simulink library "loco_native_lib"  (R2024b)
settings: Solver=VariableStepAuto  StartTime=0.0  StopTime=10.0  RelTol=1e-3
undefined symbols (not defined in the file): P, PN
libraries: fl_lib x96, nesl_utility x44, $bdroot x21, simulink x2, sdl_lib x1, batteryecm_lib x1
(part 1 of 2)
settings Model: Creator=BillBeverley  LastModifiedBy=BillBeverley

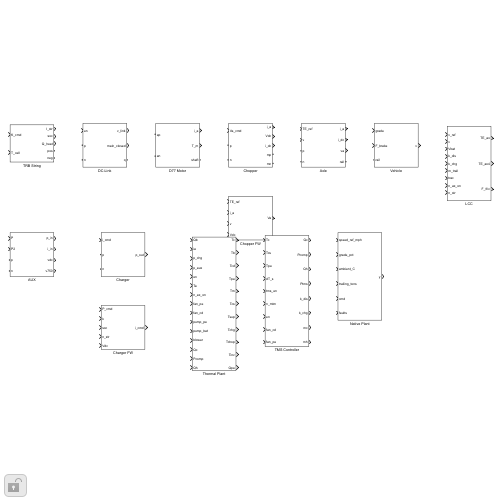
[thumbnail: Simulink's stored preview of the top-level diagram]
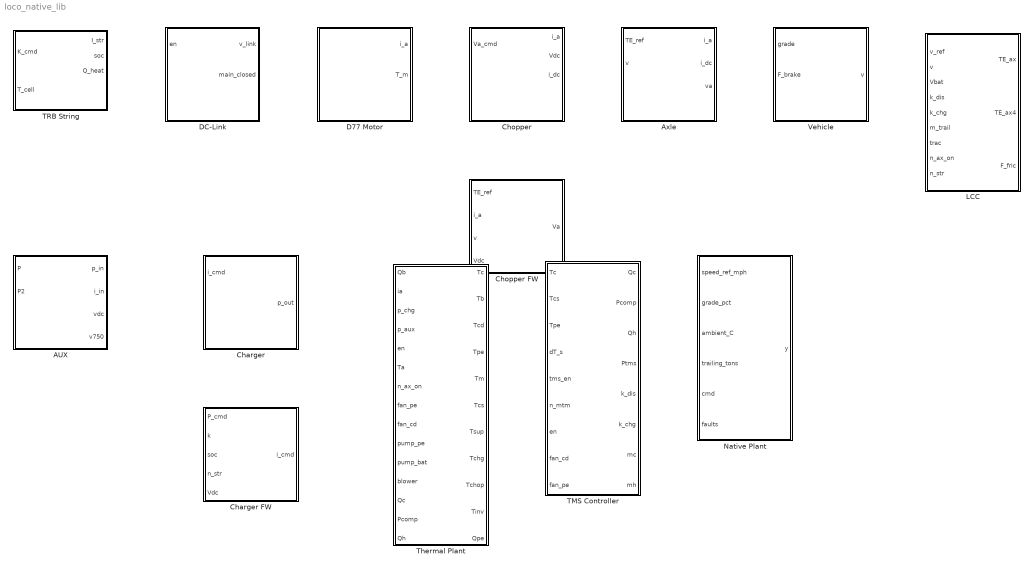
== system loco_native_lib ==
  AUX : Subsystem  mask{eta=P.aux.eta, P_max=P.aux.P_max, V750=750, V_floor=100}
      mask prompts: eta "Converter efficiency"; P_max "Max output power (W)"; V750 "AUX bus voltage (V)"; V_floor "Input voltage floor (V)"
  Axle : Subsystem
  Charger : Subsystem
  Charger FW : Subsystem  mask{P_max=P.chg.P_max, I_max=P.chg.I_hw, I_bms=P.chg.I_bms, soc_max=P.chg.soc_max, soc_band=P.chg.soc_band, V_floor=100, N_str_nom=P.batt.Np, Ts=0.01}
  Chopper : Subsystem
  Chopper FW : Subsystem  mask{A=PN.ax}
      mask prompts: A "Axle parameters (struct)"
  D77 Motor : Subsystem
  DC-Link : Subsystem
  LCC : Subsystem  mask{L=PN.lcc}
      mask prompts: L "LCC parameters (struct)"
  Native Plant : Subsystem
  TMS Controller : Subsystem  mask{TH=P.th, Ts=0.1}
      mask prompts: TH "Thermal parameters (struct)"; Ts "Controller sample time (s)"
  TRB String : Subsystem
  Thermal Plant : Subsystem  mask{TH=P.th, f_ram=0.2}
      mask prompts: TH "Thermal parameters (struct)"; f_ram "Ram-air fraction"
  Vehicle : Subsystem

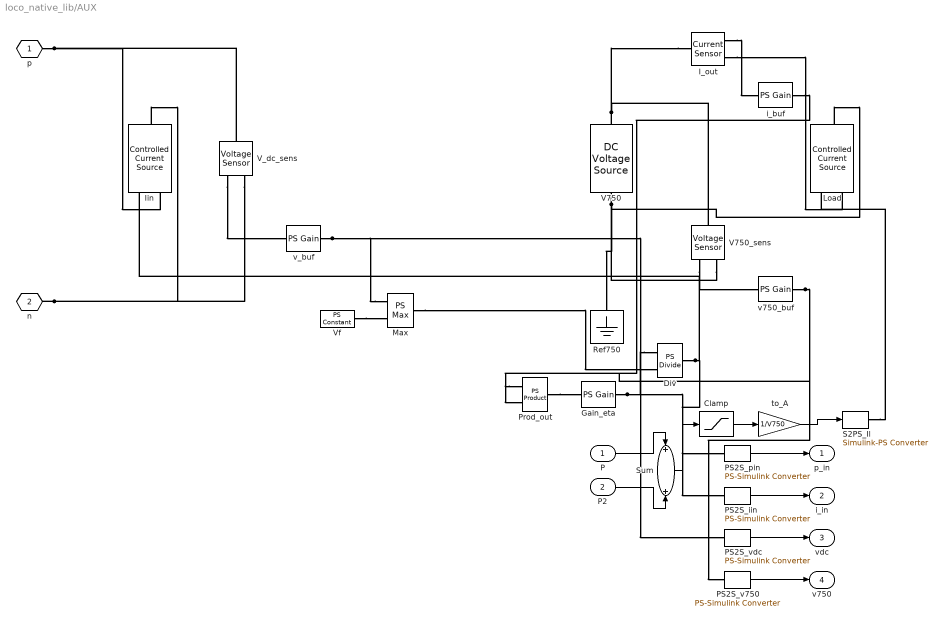
== system loco_native_lib/AUX ==
  P : Inport
  P2 : Inport  Port=2
  Clamp : Saturate  UpperLimit=P_max  LowerLimit=0
  Div : fl_lib/Physical Signals/Functions/PS Divide
  Gain_eta : fl_lib/Physical Signals/Functions/PS Gain  gain=1/eta
  I_out : fl_lib/Electrical/Electrical Sensors/Current Sensor
  Iin : fl_lib/Electrical/Electrical Sources/Controlled Current Source
  Load : fl_lib/Electrical/Electrical Sources/Controlled Current Source
  Max : fl_lib/Physical Signals/Nonlinear Operators/PS Max
      settings: InternalSimscapePortConfiguration="{\"Bottom\":[],\"Left\":[{\"id\":\"I1\",\"label\":\"\",\"type\":\"input\"},{\"id\":\"I2\",\"label\":\"\",\"type\":\"input\"}],\"Right\":[{\"id\":\"O\",\"label\":\"\",\"type\":\"output\"}],\"Top\":[]}"
  PS2S_iin : nesl_utility/PS-Simulink Converter  PhysicalDomain=network_engine_domain  SubClassName=ps_output  LeftPortType=input  RightPortType=output  PseudoPeriodic=off  Frequencies=[]  VectorFormat=inherit  Unit=A  AffineConversion=off
  PS2S_pin : nesl_utility/PS-Simulink Converter  PhysicalDomain=network_engine_domain  SubClassName=ps_output  LeftPortType=input  RightPortType=output  PseudoPeriodic=off  Frequencies=[]  VectorFormat=inherit  Unit=W  AffineConversion=off
  PS2S_v750 : nesl_utility/PS-Simulink Converter  PhysicalDomain=network_engine_domain  SubClassName=ps_output  LeftPortType=input  RightPortType=output  PseudoPeriodic=off  Frequencies=[]  VectorFormat=inherit  Unit=V  AffineConversion=off
  PS2S_vdc : nesl_utility/PS-Simulink Converter  PhysicalDomain=network_engine_domain  SubClassName=ps_output  LeftPortType=input  RightPortType=output  PseudoPeriodic=off  Frequencies=[]  VectorFormat=inherit  Unit=V  AffineConversion=off
  Prod_out : fl_lib/Physical Signals/Functions/PS Product
  Ref750 : fl_lib/Electrical/Electrical Elements/Electrical Reference
  S2PS_Il : nesl_utility/Simulink-PS Converter  PhysicalDomain=network_engine_domain  SubClassName=ps_input  LeftPortType=input  RightPortType=output  PseudoPeriodic=off  Frequencies=[]  NoiseDistribution=none  NoiseParameters=[]  Unit=A  AffineConversion=off  FilteringAndDerivatives=provide  SimscapeFilterOrder=1  InputFilterTimeConstant=0.001  UdotUserProvided=0
  Sum : Sum
  V750 : fl_lib/Electrical/Electrical Sources/DC Voltage Source  v0=V750 V
  V750_sens : fl_lib/Electrical/Electrical Sensors/Voltage Sensor
  V_dc_sens : fl_lib/Electrical/Electrical Sensors/Voltage Sensor
  Vf : fl_lib/Physical Signals/Sources/PS Constant  constant=V_floor V
  i_buf : fl_lib/Physical Signals/Functions/PS Gain  gain=1
  to_A : Gain  Gain=1/V750
  v750_buf : fl_lib/Physical Signals/Functions/PS Gain  gain=1
  v_buf : fl_lib/Physical Signals/Functions/PS Gain  gain=1
  p : PMIOPort  Side=Left
  n : PMIOPort  Port=2  Side=Left
  p_in : Outport
  i_in : Outport  Port=2
  vdc : Outport  Port=3
  v750 : Outport  Port=4
  wires:
  PS2S_pin/1 -> p_in/1
  PS2S_iin/1 -> i_in/1
  PS2S_vdc/1 -> vdc/1
  PS2S_v750/1 -> v750/1
  P/1 -> Sum/1
  P2/1 -> Sum/2
  Sum/1 -> Clamp/1
  Clamp/1 -> to_A/1
  to_A/1 -> S2PS_Il/1
  connections:
  Iin/RConn2 -- p/RConn1 -- V_dc_sens/LConn1
  n/RConn1 -- Iin/LConn1 -- V_dc_sens/RConn2
  I_out/LConn1 -- V750/LConn1 -- V750_sens/LConn1
  I_out/RConn2 -- Load/RConn2
  Load/LConn1 -- Ref750/LConn1 -- V750/RConn1 -- V750_sens/RConn2
  S2PS_Il/RConn1 -- Load/RConn1
  V_dc_sens/RConn1 -- v_buf/LConn1
  V750_sens/RConn1 -- v750_buf/LConn1
  I_out/RConn1 -- i_buf/LConn1
  Iin/RConn1 -- Div/RConn1 -- PS2S_iin/LConn1
  Prod_out/LConn1 -- v750_buf/RConn1 -- PS2S_v750/LConn1
  i_buf/RConn1 -- Prod_out/LConn2
  Prod_out/RConn1 -- Gain_eta/LConn1
  Max/LConn1 -- v_buf/RConn1 -- PS2S_vdc/LConn1
  Vf/RConn1 -- Max/LConn2
  Div/LConn1 -- Gain_eta/RConn1 -- PS2S_pin/LConn1
  Max/RConn1 -- Div/LConn2

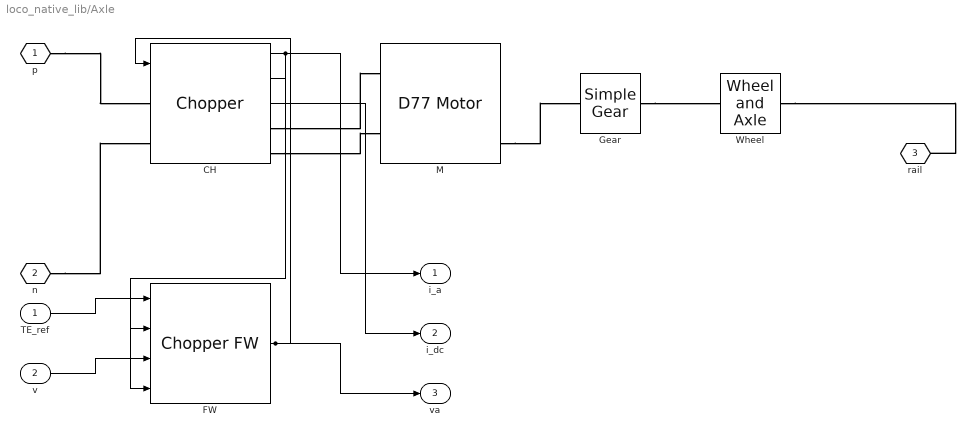
== system loco_native_lib/Axle ==
  TE_ref : Inport
  v : Inport  Port=2
  CH : $bdroot/Chopper  SystemSampleTime=-1  VariantActivationTime=update diagram  AllowFlexibleInterface=on  Latency=0  AutoFrameSizeCalculation=off
  FW : $bdroot/Chopper FW  A=PN.ax
  Gear : sdl_lib/Gears/Simple Gear  ratio=PN.ax.G  rotation_direction=sdl.enum.shaftOutputDirection.same  friction_model=sdl.enum.gear_efficiencies_load.constant  T_noload=0.1 N*m  T_nom=5 N*m  efficiency_nom=0.8  efficiency=PN.ax.eta_g  temperature_TLU=[280, 300, 320] K  load_TLU=[1, 5, 10] N*m  efficiency_TLU=[.95, .9, .85]  efficiency_TLU2=[.85, .8, .75; .95, .9, .85; .85, .8, .7]  w_thr=0.01 rad/s  pwr_thr=1e3 W  enable_backlash=false  hardstop_model=simscape.enum.hardstop.smooth  backlash_distance=1e-3 mm  r_base=0.1 m  transition=1e-4 mm  backlash_stiffness=1e6 N/m  backlash_damping=1e3 N*s/m  coeff_rest=0.7  v_tol=0.001 m/s  f_tol=0.001 N  mu_visc=[0, 0] N*m*s/rad  thermal_mass=50 J/K  temperature_specify=off  temperature_priority=High  temperature=300 K  temperature_nominal_specify=off  temperature_nominal_value=1  temperature_nominal_unit=K  x_backlash_specify=off  x_backlash_priority=None  x_backlash=0 mm  x_backlash_nominal_specify=off  x_backlash_nominal_value=1  x_backlash_nominal_unit=mm  f_hardstop_specify=off  f_hardstop_priority=None  f_hardstop=0 N  f_hardstop_nominal_specify=off  f_hardstop_nominal_value=1  f_hardstop_nominal_unit=N  v_backlash_specify=off  v_backlash_priority=None  v_backlash=0 m/s  v_backlash_nominal_specify=off  v_backlash_nominal_value=1  v_backlash_nominal_unit=m/s
  M : $bdroot/D77 Motor  SystemSampleTime=-1  VariantActivationTime=update diagram  AllowFlexibleInterface=on  Latency=0  AutoFrameSizeCalculation=off
  Wheel : fl_lib/Mechanical/Mechanisms/Wheel and Axle  R=PN.ax.r_w m  or=1  t_specify=off  t_priority=None  t=0 N*m  t_nominal_specify=off  t_nominal_value=1  t_nominal_unit=N*m  f_specify=off  f_priority=None  f=0 N  f_nominal_specify=off  f_nominal_value=1  f_nominal_unit=N
  p : PMIOPort  Side=Left
  n : PMIOPort  Port=2  Side=Left
  rail : PMIOPort  Port=3  Side=Right
  i_a : Outport
  i_dc : Outport  Port=2
  va : Outport  Port=3
  wires:
  TE_ref/1 -> FW/1
  CH/1 -> FW/2, i_a/1
  v/1 -> FW/3
  CH/2 -> FW/4
  FW/1 -> CH/1, va/1
  CH/3 -> i_dc/1
  connections:
  p/RConn1 -- CH/LConn1
  n/RConn1 -- CH/LConn2
  CH/RConn1 -- M/LConn1
  CH/RConn2 -- M/LConn2
  M/RConn1 -- Gear/LConn1
  Gear/RConn1 -- Wheel/LConn1
  Wheel/RConn1 -- rail/RConn1

== system loco_native_lib/Charger ==
  i_cmd : Inport
  Ichg : fl_lib/Electrical/Electrical Sources/Controlled Current Source
  PS2S_p : nesl_utility/PS-Simulink Converter  PhysicalDomain=network_engine_domain  SubClassName=ps_output  LeftPortType=input  RightPortType=output  PseudoPeriodic=off  Frequencies=[]  VectorFormat=inherit  Unit=W  AffineConversion=off
  Prod : fl_lib/Physical Signals/Functions/PS Product
  S2PS_i : nesl_utility/Simulink-PS Converter  PhysicalDomain=network_engine_domain  SubClassName=ps_input  LeftPortType=input  RightPortType=output  PseudoPeriodic=off  Frequencies=[]  NoiseDistribution=none  NoiseParameters=[]  Unit=A  AffineConversion=off  FilteringAndDerivatives=provide  SimscapeFilterOrder=1  InputFilterTimeConstant=0.001  UdotUserProvided=0
  V_sens : fl_lib/Electrical/Electrical Sensors/Voltage Sensor
  p : PMIOPort  Side=Left
  n : PMIOPort  Port=2  Side=Left
  p_out : Outport
  wires:
  i_cmd/1 -> S2PS_i/1
  PS2S_p/1 -> p_out/1
  connections:
  p/RConn1 -- Ichg/LConn1 -- V_sens/LConn1
  n/RConn1 -- Ichg/RConn2 -- V_sens/RConn2
  Ichg/RConn1 -- S2PS_i/RConn1 -- Prod/LConn1
  V_sens/RConn1 -- Prod/LConn2
  Prod/RConn1 -- PS2S_p/LConn1

== system loco_native_lib/Charger FW ==
  P_cmd : Inport
  k : Inport  Port=2
  soc : Inport  Port=3
  n_str : Inport  Port=4
  Vdc : Inport  Port=5
  Mux : Mux  Inputs=5
  Sample : ZeroOrderHold  SampleTime=Ts
  Scan : UnitDelay  SampleTime=Ts  HasFrameUpgradeWarning=on
  chg : MATLAB Function  TreatAsAtomicUnit=on
  i_cmd : Outport
  wires:
  P_cmd/1 -> Mux/1
  k/1 -> Mux/2
  soc/1 -> Mux/3
  n_str/1 -> Mux/4
  Vdc/1 -> Mux/5
  Mux/1 -> Sample/1
  Sample/1 -> chg/1(u)
  chg/1(i) -> Scan/1
  Scan/1 -> i_cmd/1

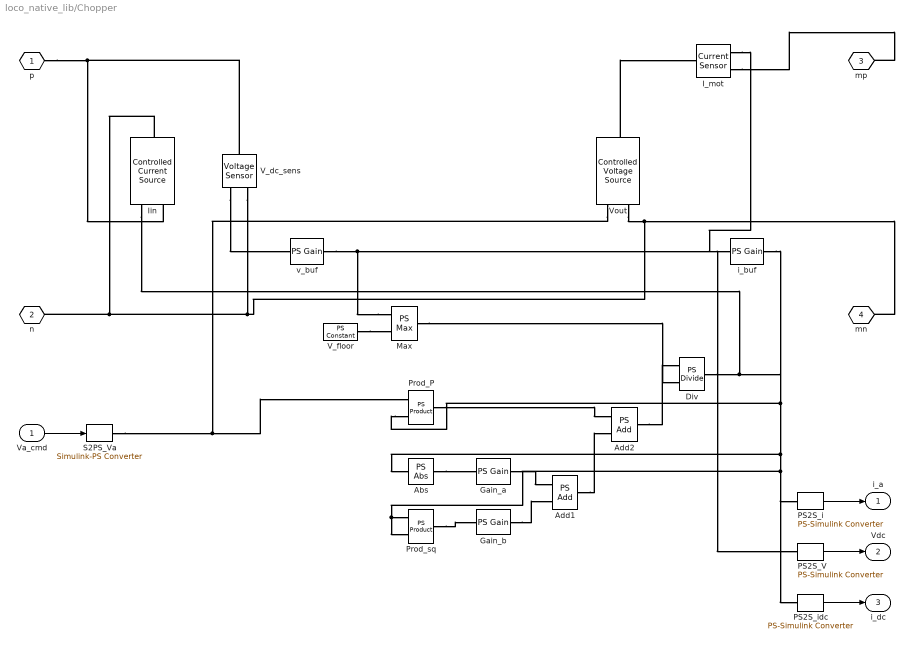
== system loco_native_lib/Chopper ==
  Va_cmd : Inport
  Abs : fl_lib/Physical Signals/Nonlinear Operators/PS Abs
      settings: InternalSimscapePortConfiguration="{\"Bottom\":[],\"Left\":[{\"id\":\"I\",\"label\":\"\",\"type\":\"input\"}],\"Right\":[{\"id\":\"O\",\"label\":\"\",\"type\":\"output\"}],\"Top\":[]}"
  Add1 : fl_lib/Physical Signals/Functions/PS Add
  Add2 : fl_lib/Physical Signals/Functions/PS Add
  Div : fl_lib/Physical Signals/Functions/PS Divide
  Gain_a : fl_lib/Physical Signals/Functions/PS Gain  gain=PN.ax.a_loss V
  Gain_b : fl_lib/Physical Signals/Functions/PS Gain  gain=PN.ax.b_loss Ohm
  I_mot : fl_lib/Electrical/Electrical Sensors/Current Sensor
  Iin : fl_lib/Electrical/Electrical Sources/Controlled Current Source
  Max : fl_lib/Physical Signals/Nonlinear Operators/PS Max
      settings: InternalSimscapePortConfiguration="{\"Bottom\":[],\"Left\":[{\"id\":\"I1\",\"label\":\"\",\"type\":\"input\"},{\"id\":\"I2\",\"label\":\"\",\"type\":\"input\"}],\"Right\":[{\"id\":\"O\",\"label\":\"\",\"type\":\"output\"}],\"Top\":[]}"
  PS2S_V : nesl_utility/PS-Simulink Converter  PhysicalDomain=network_engine_domain  SubClassName=ps_output  LeftPortType=input  RightPortType=output  PseudoPeriodic=off  Frequencies=[]  VectorFormat=inherit  Unit=V  AffineConversion=off
  PS2S_i : nesl_utility/PS-Simulink Converter  PhysicalDomain=network_engine_domain  SubClassName=ps_output  LeftPortType=input  RightPortType=output  PseudoPeriodic=off  Frequencies=[]  VectorFormat=inherit  Unit=A  AffineConversion=off
  PS2S_idc : nesl_utility/PS-Simulink Converter  PhysicalDomain=network_engine_domain  SubClassName=ps_output  LeftPortType=input  RightPortType=output  PseudoPeriodic=off  Frequencies=[]  VectorFormat=inherit  Unit=A  AffineConversion=off
  Prod_P : fl_lib/Physical Signals/Functions/PS Product
  Prod_sq : fl_lib/Physical Signals/Functions/PS Product
  S2PS_Va : nesl_utility/Simulink-PS Converter  PhysicalDomain=network_engine_domain  SubClassName=ps_input  LeftPortType=input  RightPortType=output  PseudoPeriodic=off  Frequencies=[]  NoiseDistribution=none  NoiseParameters=[]  Unit=V  AffineConversion=off  FilteringAndDerivatives=filter  SimscapeFilterOrder=1  InputFilterTimeConstant=1e-4  UdotUserProvided=0
  V_dc_sens : fl_lib/Electrical/Electrical Sensors/Voltage Sensor
  V_floor : fl_lib/Physical Signals/Sources/PS Constant  constant=PN.ax.V_floor V
  Vout : fl_lib/Electrical/Electrical Sources/Controlled Voltage Source
  i_buf : fl_lib/Physical Signals/Functions/PS Gain  gain=1
  v_buf : fl_lib/Physical Signals/Functions/PS Gain  gain=1
  p : PMIOPort  Side=Left
  n : PMIOPort  Port=2  Side=Left
  mp : PMIOPort  Port=3  Side=Right
  mn : PMIOPort  Port=4  Side=Right
  i_a : Outport
  Vdc : Outport  Port=2
  i_dc : Outport  Port=3
  wires:
  Va_cmd/1 -> S2PS_Va/1
  PS2S_i/1 -> i_a/1
  PS2S_V/1 -> Vdc/1
  PS2S_idc/1 -> i_dc/1
  connections:
  S2PS_Va/RConn1 -- Vout/RConn1 -- Prod_P/LConn1
  Prod_P/LConn2 -- i_buf/RConn1 -- Prod_sq/LConn1 -- Prod_sq/LConn2 -- PS2S_i/LConn1 -- Abs/LConn1
  Abs/RConn1 -- Gain_a/LConn1
  Prod_sq/RConn1 -- Gain_b/LConn1
  Gain_a/RConn1 -- Add1/LConn1
  Gain_b/RConn1 -- Add1/LConn2
  Prod_P/RConn1 -- Add2/LConn1
  Add1/RConn1 -- Add2/LConn2
  Max/LConn1 -- v_buf/RConn1 -- PS2S_V/LConn1
  V_floor/RConn1 -- Max/LConn2
  Add2/RConn1 -- Div/LConn1
  Max/RConn1 -- Div/LConn2
  Div/RConn1 -- Iin/RConn1 -- PS2S_idc/LConn1
  p/RConn1 -- V_dc_sens/LConn1 -- Iin/RConn2
  Vout/RConn2 -- n/RConn1 -- Iin/LConn1 -- V_dc_sens/RConn2 -- mn/RConn1
  Vout/LConn1 -- I_mot/LConn1
  I_mot/RConn2 -- mp/RConn1
  I_mot/RConn1 -- i_buf/LConn1
  V_dc_sens/RConn1 -- v_buf/LConn1

== system loco_native_lib/Chopper FW ==
  TE_ref : Inport
  i_a : Inport  Port=2
  v : Inport  Port=3
  Vdc : Inport  Port=4
  Scan : UnitDelay  SampleTime=A.Ts_fw  HasFrameUpgradeWarning=on
  fw : MATLAB Function  TreatAsAtomicUnit=on
  Va : Outport
  wires:
  TE_ref/1 -> fw/1(TE_ref)
  i_a/1 -> fw/2(i_a)
  v/1 -> fw/3(v)
  Vdc/1 -> fw/4(Vdc)
  fw/1(Va) -> Scan/1
  Scan/1 -> Va/1

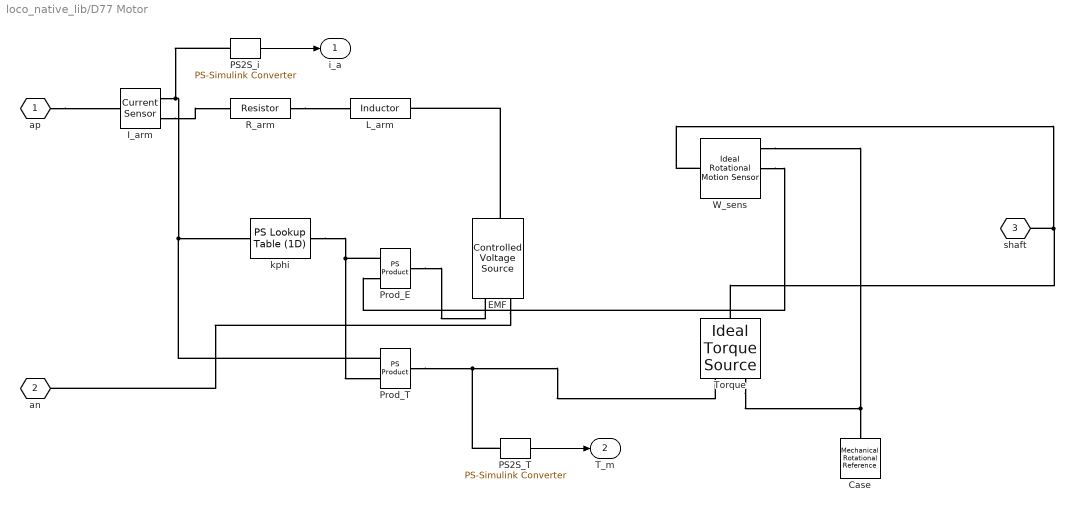
== system loco_native_lib/D77 Motor ==
  Case : fl_lib/Mechanical/Rotational Elements/Mechanical Rotational Reference
  EMF : fl_lib/Electrical/Electrical Sources/Controlled Voltage Source
  I_arm : fl_lib/Electrical/Electrical Sensors/Current Sensor
  L_arm : fl_lib/Electrical/Electrical Elements/Inductor  l=PN.ax.L_a H  r=0 Ohm  g=1e-9 1/Ohm  i_specify=off  i_priority=None  i=0 A  i_nominal_specify=off  i_nominal_value=1  i_nominal_unit=A  v_specify=off  v_priority=None  v=0 V  v_nominal_specify=off  v_nominal_value=1  v_nominal_unit=V  i_L_specify=off  i_L_priority=High  i_L=0 A  i_L_nominal_specify=off  i_L_nominal_value=1  i_L_nominal_unit=A
  PS2S_T : nesl_utility/PS-Simulink Converter  PhysicalDomain=network_engine_domain  SubClassName=ps_output  LeftPortType=input  RightPortType=output  PseudoPeriodic=off  Frequencies=[]  VectorFormat=inherit  Unit=N*m  AffineConversion=off
  PS2S_i : nesl_utility/PS-Simulink Converter  PhysicalDomain=network_engine_domain  SubClassName=ps_output  LeftPortType=input  RightPortType=output  PseudoPeriodic=off  Frequencies=[]  VectorFormat=inherit  Unit=A  AffineConversion=off
  Prod_E : fl_lib/Physical Signals/Functions/PS Product
  Prod_T : fl_lib/Physical Signals/Functions/PS Product
  R_arm : fl_lib/Electrical/Electrical Elements/Resistor  R=PN.ax.R_m Ohm  i_specify=off  i_priority=None  i=0 A  i_nominal_specify=off  i_nominal_value=1  i_nominal_unit=A  v_specify=off  v_priority=None  v=0 V  v_nominal_specify=off  v_nominal_value=1  v_nominal_unit=V
  Torque : fl_lib/Mechanical/Mechanical Sources/Ideal Torque Source
  W_sens : fl_lib/Mechanical/Mechanical Sensors/Ideal Rotational Motion Sensor  reference=foundation.enum.MeasurementReference.difference  acceleration_port=false  velocity_port=true  position_port=true  wrap_angle=false  offset=0 rad
  kphi : fl_lib/Physical Signals/Lookup Tables/PS Lookup Table (1D)  x=PN.ax.i_k A  f=PN.ax.kphi_k V*s/rad  interp_method=simscape.enum.interpolation.linear  extrap_method=simscape.enum.extrapolation.linear
  ap : PMIOPort  Side=Left
  an : PMIOPort  Port=2  Side=Left
  shaft : PMIOPort  Port=3  Side=Right
  i_a : Outport
  T_m : Outport  Port=2
  wires:
  PS2S_i/1 -> i_a/1
  PS2S_T/1 -> T_m/1
  connections:
  ap/RConn1 -- I_arm/LConn1
  I_arm/RConn2 -- R_arm/LConn1
  R_arm/RConn1 -- L_arm/LConn1
  EMF/LConn1 -- L_arm/RConn1
  EMF/RConn2 -- an/RConn1
  Torque/LConn1 -- W_sens/LConn1 -- shaft/RConn1
  Torque/RConn2 -- Case/LConn1 -- W_sens/RConn1
  I_arm/RConn1 -- PS2S_i/LConn1 -- Prod_T/LConn1 -- kphi/LConn1
  kphi/RConn1 -- Prod_E/LConn1 -- Prod_T/LConn2
  W_sens/RConn2 -- Prod_E/LConn2
  Prod_E/RConn1 -- EMF/RConn1
  Prod_T/RConn1 -- PS2S_T/LConn1 -- Torque/RConn1

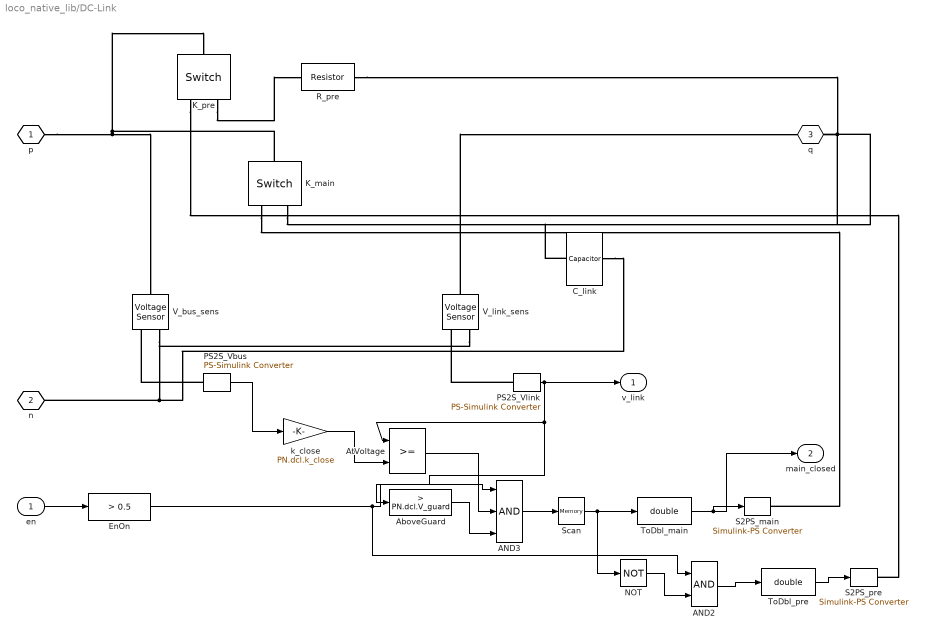
== system loco_native_lib/DC-Link ==
  en : Inport
  AND2 : Logic  AllPortsSameDT=off  OutDataTypeStr=boolean
  AND3 : Logic  Inputs=3  AllPortsSameDT=off  OutDataTypeStr=boolean
  AboveGuard : simulink/Logic and Bit Operations/Compare To Constant  relop=>  const=PN.dcl.V_guard  OutDataTypeStr=boolean
  AtVoltage : RelationalOperator  OutDataTypeStr=boolean  RndMeth=Simplest  InputSameDT=off
  C_link : fl_lib/Electrical/Electrical Elements/Capacitor  c=PN.dcl.C F  r=1e-6 Ohm  g=0 1/Ohm  i_specify=off  i_priority=None  i=0 A  i_nominal_specify=off  i_nominal_value=1  i_nominal_unit=A  v_specify=off  v_priority=None  v=0 V  v_nominal_specify=off  v_nominal_value=1  v_nominal_unit=V  vc_specify=off  vc_priority=High  vc=0 V  vc_nominal_specify=off  vc_nominal_value=1  vc_nominal_unit=V
  EnOn : simulink/Logic and Bit Operations/Compare To Constant  relop=>  const=0.5  OutDataTypeStr=boolean
  K_main : fl_lib/Electrical/Electrical Elements/Switch  R_closed=PN.dcl.R_on Ohm  G_open=1e-9 1/Ohm  Threshold=0.5  i_specify=off  i_priority=None  i=0 A  i_nominal_specify=off  i_nominal_value=1  i_nominal_unit=A  v_specify=off  v_priority=None  v=0 V  v_nominal_specify=off  v_nominal_value=1  v_nominal_unit=V
  K_pre : fl_lib/Electrical/Electrical Elements/Switch  R_closed=PN.dcl.R_pre_k Ohm  G_open=1e-9 1/Ohm  Threshold=0.5  i_specify=off  i_priority=None  i=0 A  i_nominal_specify=off  i_nominal_value=1  i_nominal_unit=A  v_specify=off  v_priority=None  v=0 V  v_nominal_specify=off  v_nominal_value=1  v_nominal_unit=V
  NOT : Logic  Operator=NOT  AllPortsSameDT=off  OutDataTypeStr=boolean
  PS2S_Vbus : nesl_utility/PS-Simulink Converter  PhysicalDomain=network_engine_domain  SubClassName=ps_output  LeftPortType=input  RightPortType=output  PseudoPeriodic=off  Frequencies=[]  VectorFormat=inherit  Unit=V  AffineConversion=off
  PS2S_Vlink : nesl_utility/PS-Simulink Converter  PhysicalDomain=network_engine_domain  SubClassName=ps_output  LeftPortType=input  RightPortType=output  PseudoPeriodic=off  Frequencies=[]  VectorFormat=inherit  Unit=V  AffineConversion=off
  R_pre : fl_lib/Electrical/Electrical Elements/Resistor  R=PN.dcl.R_pre Ohm  i_specify=off  i_priority=None  i=0 A  i_nominal_specify=off  i_nominal_value=1  i_nominal_unit=A  v_specify=off  v_priority=None  v=0 V  v_nominal_specify=off  v_nominal_value=1  v_nominal_unit=V
  S2PS_main : nesl_utility/Simulink-PS Converter  PhysicalDomain=network_engine_domain  SubClassName=ps_input  LeftPortType=input  RightPortType=output  PseudoPeriodic=off  Frequencies=[]  NoiseDistribution=none  NoiseParameters=[]  Unit=1  AffineConversion=off  FilteringAndDerivatives=provide  SimscapeFilterOrder=1  InputFilterTimeConstant=0.001  UdotUserProvided=0
  S2PS_pre : nesl_utility/Simulink-PS Converter  PhysicalDomain=network_engine_domain  SubClassName=ps_input  LeftPortType=input  RightPortType=output  PseudoPeriodic=off  Frequencies=[]  NoiseDistribution=none  NoiseParameters=[]  Unit=1  AffineConversion=off  FilteringAndDerivatives=provide  SimscapeFilterOrder=1  InputFilterTimeConstant=0.001  UdotUserProvided=0
  Scan : Memory
  ToDbl_main : DataTypeConversion  OutDataTypeStr=double  SaturateOnIntegerOverflow=off  RndMeth=Floor
  ToDbl_pre : DataTypeConversion  OutDataTypeStr=double  SaturateOnIntegerOverflow=off  RndMeth=Floor
  V_bus_sens : fl_lib/Electrical/Electrical Sensors/Voltage Sensor
  V_link_sens : fl_lib/Electrical/Electrical Sensors/Voltage Sensor
  k_close : Gain  Gain=PN.dcl.k_close
  p : PMIOPort  Side=Left
  n : PMIOPort  Port=2  Side=Left
  q : PMIOPort  Port=3  Side=Right
  v_link : Outport
  main_closed : Outport  Port=2
  wires:
  en/1 -> EnOn/1
  EnOn/1 -> AND3/1, AND2/1
  PS2S_Vlink/1 -> AtVoltage/1, AboveGuard/1, v_link/1
  PS2S_Vbus/1 -> k_close/1
  k_close/1 -> AtVoltage/2
  AtVoltage/1 -> AND3/2
  AboveGuard/1 -> AND3/3
  AND3/1 -> Scan/1
  Scan/1 -> ToDbl_main/1, NOT/1
  ToDbl_main/1 -> S2PS_main/1, main_closed/1
  NOT/1 -> AND2/2
  AND2/1 -> ToDbl_pre/1
  ToDbl_pre/1 -> S2PS_pre/1
  connections:
  R_pre/RConn1 -- q/RConn1 -- K_main/RConn2 -- V_link_sens/LConn1 -- C_link/LConn1
  p/RConn1 -- V_bus_sens/LConn1 -- K_main/LConn1 -- K_pre/LConn1
  K_pre/RConn2 -- R_pre/LConn1
  C_link/RConn1 -- V_link_sens/RConn2 -- V_bus_sens/RConn2 -- n/RConn1
  K_pre/RConn1 -- S2PS_pre/RConn1
  K_main/RConn1 -- S2PS_main/RConn1
  PS2S_Vlink/LConn1 -- V_link_sens/RConn1
  PS2S_Vbus/LConn1 -- V_bus_sens/RConn1

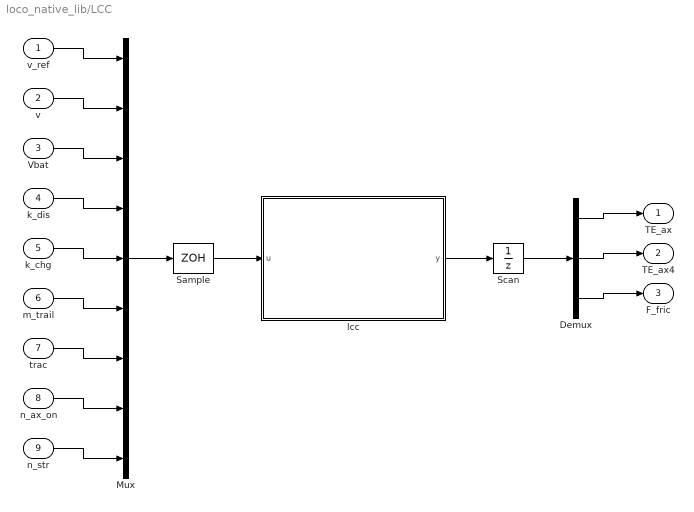
== system loco_native_lib/LCC ==
  v_ref : Inport
  v : Inport  Port=2
  Vbat : Inport  Port=3
  k_dis : Inport  Port=4
  k_chg : Inport  Port=5
  m_trail : Inport  Port=6
  trac : Inport  Port=7
  n_ax_on : Inport  Port=8
  n_str : Inport  Port=9
  Demux : Demux  Outputs=3
  Mux : Mux  Inputs=9
  Sample : ZeroOrderHold  SampleTime=PN.lcc.Ts
  Scan : UnitDelay  SampleTime=PN.lcc.Ts  HasFrameUpgradeWarning=on
  lcc : MATLAB Function  TreatAsAtomicUnit=on
  TE_ax : Outport
  TE_ax4 : Outport  Port=2
  F_fric : Outport  Port=3
  wires:
  v_ref/1 -> Mux/1
  v/1 -> Mux/2
  Vbat/1 -> Mux/3
  k_dis/1 -> Mux/4
  k_chg/1 -> Mux/5
  m_trail/1 -> Mux/6
  trac/1 -> Mux/7
  n_ax_on/1 -> Mux/8
  n_str/1 -> Mux/9
  Mux/1 -> Sample/1
  Sample/1 -> lcc/1(u)
  lcc/1(y) -> Scan/1
  Scan/1 -> Demux/1
  Demux/1 -> TE_ax/1
  Demux/2 -> TE_ax4/1
  Demux/3 -> F_fric/1

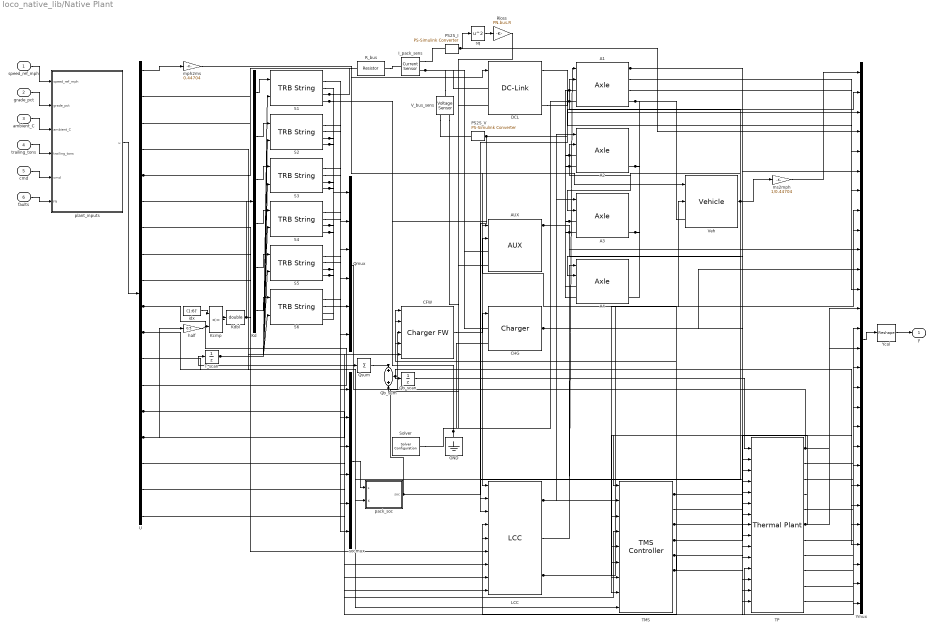
== system loco_native_lib/Native Plant ==
  speed_ref_mph : Inport
  grade_pct : Inport  Port=2
  ambient_C : Inport  Port=3
  trailing_tons : Inport  Port=4
  cmd : Inport  Port=5
  faults : Inport  Port=6
  A{1..4} (4 alike) : $bdroot/Axle  SystemSampleTime=-1  VariantActivationTime=update diagram  AllowFlexibleInterface=on  Latency=0  AutoFrameSizeCalculation=off
  AUX : $bdroot/AUX  eta=P.aux.eta  P_max=P.aux.P_max  V750=750  V_floor=100
  CFW : $bdroot/Charger FW  P_max=P.chg.P_max  I_max=P.chg.I_hw  I_bms=P.chg.I_bms  soc_max=P.chg.soc_max  soc_band=P.chg.soc_band  V_floor=100  N_str_nom=P.batt.Np  Ts=0.01
  CHG : $bdroot/Charger  SystemSampleTime=-1  VariantActivationTime=update diagram  AllowFlexibleInterface=on  Latency=0  AutoFrameSizeCalculation=off
  DCL : $bdroot/DC-Link  SystemSampleTime=-1  VariantActivationTime=update diagram  AllowFlexibleInterface=on  Latency=0  AutoFrameSizeCalculation=off
  GND : fl_lib/Electrical/Electrical Elements/Electrical Reference
  I_pack_sens : fl_lib/Electrical/Electrical Sensors/Current Sensor
  Kcmp : RelationalOperator  Operator=<=  OutDataTypeStr=boolean  RndMeth=Simplest  InputSameDT=off
  Kd : Demux  Outputs=6
  Kdbl : DataTypeConversion  OutDataTypeStr=double  SaturateOnIntegerOverflow=off  RndMeth=Floor
  LCC : $bdroot/LCC  L=PN.lcc
  PS2S_I : nesl_utility/PS-Simulink Converter  PhysicalDomain=network_engine_domain  SubClassName=ps_output  LeftPortType=input  RightPortType=output  PseudoPeriodic=off  Frequencies=[]  VectorFormat=inherit  Unit=A  AffineConversion=off
  PS2S_V : nesl_utility/PS-Simulink Converter  PhysicalDomain=network_engine_domain  SubClassName=ps_output  LeftPortType=input  RightPortType=output  PseudoPeriodic=off  Frequencies=[]  VectorFormat=inherit  Unit=V  AffineConversion=off
  Qb_scan : UnitDelay  SampleTime=0.1  HasFrameUpgradeWarning=on
  Qb_sum : Sum
  Qmux : Mux  Inputs=6
  Qsum : Sum  Inputs=+
  R_bus : fl_lib/Electrical/Electrical Elements/Resistor  R=PN.bus.R Ohm  i_specify=off  i_priority=None  i=0 A  i_nominal_specify=off  i_nominal_value=1  i_nominal_unit=A  v_specify=off  v_priority=None  v=0 V  v_nominal_specify=off  v_nominal_value=1  v_nominal_unit=V
  Rloss : Gain  Gain=PN.bus.R
  S{1..6} (6 alike) : $bdroot/TRB String  SystemSampleTime=-1  VariantActivationTime=update diagram  AllowFlexibleInterface=on  Latency=0  AutoFrameSizeCalculation=off
  Solver : nesl_utility/Solver Configuration  PhysicalDomain=network_engine_domain  SubClassName=solver  LeftPortType=input  RightPortType=generic  Tones=[]  Harmonics=[]  SimulateNoise=off  Profile=off  UseLocalSampling=off  EnableSwitchedLinearOptims=on  FrequencyDomain=off  UseCCode=off  RelTol=0.001  AbsTol=0.001  MinStep=1e-09  ToWorkspace=off  RevertToSquareIcSolve=off  NumHomotopyIterations=100  PhasorMode=off  PhasorModeNumHarmonics=1  ConsistencySolver=NEWTON_XTOL_AFTER_FTOL  IndexReductionMethod=DerivativeReplacement  DoDC=off  ResidualTolerance=1e-09  ConsistencyTolSource=GLOBAL  ConsistencyAbsTol=0.001  ConsistencyRelTol=0.001  ConsistencyTolFactor=0.001  UseLocalSolver=off  LocalSolverChoice=NE_BACKWARD_EULER_ADVANCER  ResolveIndetEquations=on  FunctionEvalNumThread=1  LocalSolverSampleTime=0.001  DoFixedCost=off  MaxNonlinIter=3  MaxModeIter=2  ComputeImpulses=off  ImpulseIterations=2  LinearAlgebra=auto  LinearAlgebraNumThread=0  EquationFormulation=NE_TIME_EF  DelaysMemoryBudget=1024  AutomaticFiltering=on  FilteringTimeConstant=0.001  PartitionStorageMethod=AS_NEEDED  PartitionMemoryBudget=1024  PartitionMethod=ROBUST  MultibodyUseLocalSolver=off  MultibodyLocalSolverChoice=ODE1  MultibodyLocalSolverSampleTime=0.001
  TMS : $bdroot/TMS Controller  TH=P.th  Ts=0.1
  TP : $bdroot/Thermal Plant  TH=P.th  f_ram=0.2
  T_scan : UnitDelay  InitialCondition=P.th.T0_bat  SampleTime=0.1  HasFrameUpgradeWarning=on
  U : Demux  Outputs=18
  V_bus_sens : fl_lib/Electrical/Electrical Sensors/Voltage Sensor
  Veh : $bdroot/Vehicle  SystemSampleTime=-1  VariantActivationTime=update diagram  AllowFlexibleInterface=on  Latency=0  AutoFrameSizeCalculation=off
  Ycol : Reshape  OutputDimensionality=Column vector (2-D)
  Ymux : Mux  Inputs=28
  half : Gain  Gain=0.5
  idx : Constant  Value=(1:6)'
  mph2ms : Gain  Gain=0.44704
  ms2mph : Gain  Gain=1/0.44704
  pack_soc : MATLAB Function  TreatAsAtomicUnit=on
  plant_inputs : MATLAB Function  TreatAsAtomicUnit=on
  socmux : Mux  Inputs=6
  sq : Math  Operator=square
  y : Outport
  wires:
  speed_ref_mph/1 -> plant_inputs/1(speed_ref_mph)
  grade_pct/1 -> plant_inputs/2(grade_pct)
  ambient_C/1 -> plant_inputs/3(ambient_C)
  trailing_tons/1 -> plant_inputs/4(trailing_tons)
  cmd/1 -> plant_inputs/5(cmd)
  faults/1 -> plant_inputs/6(flt)
  plant_inputs/1(u) -> U/1
  U/1 -> mph2ms/1
  mph2ms/1 -> LCC/1
  Veh/1 -> LCC/2, ms2mph/1, A1/2, A2/2, A3/2, A4/2
  PS2S_V/1 -> LCC/3, CFW/5, Ymux/3
  TMS/5 -> LCC/4, Ymux/27
  TMS/6 -> LCC/5, CFW/2, Ymux/28
  U/7 -> LCC/6
  U/18 -> LCC/7
  U/14 -> LCC/8, TP/7
  U/15 -> LCC/9, CFW/4, half/1
  LCC/1 -> A1/1, A2/1, A3/1, Ymux/8
  LCC/2 -> A4/1
  LCC/3 -> Veh/2, Ymux/9
  U/2 -> Veh/1
  U/5 -> DCL/1, TP/5, TMS/7
  U/3 -> AUX/1
  TMS/4 -> AUX/2, Ymux/22
  U/4 -> CFW/1
  pack_soc/1(soc) -> CFW/3, Ymux/2
  CFW/1 -> CHG/1
  Qb_scan/1 -> TP/1
  A1/1 -> TP/2, Ymux/6
  CHG/1 -> TP/3, Ymux/11
  AUX/1 -> TP/4, Ymux/10
  U/6 -> TP/6
  U/10 -> TP/8, TMS/9
  U/11 -> TP/9, TMS/8
  U/12 -> TP/10
  U/13 -> TP/11
  U/17 -> TP/12
  TMS/1 -> TP/13, Ymux/23
  TMS/2 -> TP/14
  TMS/3 -> TP/15, Ymux/24
  TP/1 -> TMS/1, T_scan/1, Ymux/13
  TP/6 -> TMS/2, Ymux/15
  TP/4 -> TMS/3
  U/16 -> TMS/4
  U/8 -> TMS/5
  U/9 -> TMS/6
  idx/1 -> Kcmp/1
  half/1 -> Kcmp/2
  Kcmp/1 -> Kdbl/1
  Kdbl/1 -> Kd/1, pack_soc/2(K)
  socmux/1 -> pack_soc/1(s)
  Qmux/1 -> Qsum/1
  Qsum/1 -> Qb_sum/1
  PS2S_I/1 -> sq/1, Ymux/4
  sq/1 -> Rloss/1
  Rloss/1 -> Qb_sum/2
  Qb_sum/1 -> Qb_scan/1, Ymux/25
  Ymux/1 -> Ycol/1
  Ycol/1 -> y/1
  Kd/1 -> S1/1
  T_scan/1 -> S1/2, S2/2, S3/2, S4/2, S5/2, S6/2
  S1/3 -> Qmux/1
  S1/2 -> socmux/1
  Kd/2 -> S2/1
  S2/3 -> Qmux/2
  S2/2 -> socmux/2
  Kd/3 -> S3/1
  S3/3 -> Qmux/3
  S3/2 -> socmux/3
  Kd/4 -> S4/1
  S4/3 -> Qmux/4
  S4/2 -> socmux/4
  Kd/5 -> S5/1
  S5/3 -> Qmux/5
  S5/2 -> socmux/5
  Kd/6 -> S6/1
  S6/3 -> Qmux/6
  S6/2 -> socmux/6
  ms2mph/1 -> Ymux/1
  DCL/1 -> Ymux/5
  A1/3 -> Ymux/7
  A1/2 -> Ymux/12
  TP/2 -> Ymux/14
  TP/3 -> Ymux/16
  TP/7 -> Ymux/17
  TP/8 -> Ymux/18
  TP/9 -> Ymux/19
  TP/10 -> Ymux/20
  TP/5 -> Ymux/21
  TP/11 -> Ymux/26
  connections:
  R_bus/LConn1 -- S1/RConn1 -- S2/RConn1 -- S3/RConn1 -- S4/RConn1 -- S5/RConn1 -- S6/RConn1
  R_bus/RConn1 -- I_pack_sens/LConn1
  V_bus_sens/LConn1 -- I_pack_sens/RConn2 -- DCL/LConn1 -- AUX/LConn1 -- CHG/LConn1
  V_bus_sens/RConn2 -- S1/RConn2 -- S2/RConn2 -- S3/RConn2 -- S4/RConn2 -- S5/RConn2 -- S6/RConn2 -- DCL/LConn2 -- AUX/LConn2 -- CHG/LConn2 -- Solver/RConn1 -- GND/LConn1 -- A1/LConn2 -- A2/LConn2 -- A3/LConn2 -- A4/LConn2
  I_pack_sens/RConn1 -- PS2S_I/LConn1
  V_bus_sens/RConn1 -- PS2S_V/LConn1
  A1/LConn1 -- DCL/RConn1 -- A2/LConn1 -- A3/LConn1 -- A4/LConn1
  Veh/LConn1 -- A1/RConn1 -- A2/RConn1 -- A3/RConn1 -- A4/RConn1

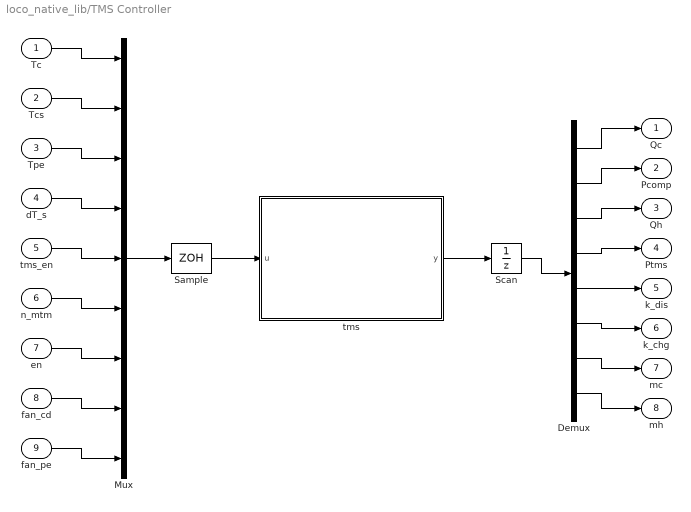
== system loco_native_lib/TMS Controller ==
  Tc : Inport
  Tcs : Inport  Port=2
  Tpe : Inport  Port=3
  dT_s : Inport  Port=4
  tms_en : Inport  Port=5
  n_mtm : Inport  Port=6
  en : Inport  Port=7
  fan_cd : Inport  Port=8
  fan_pe : Inport  Port=9
  Demux : Demux  Outputs=8
  Mux : Mux  Inputs=9
  Sample : ZeroOrderHold  SampleTime=Ts
  Scan : UnitDelay  SampleTime=Ts  HasFrameUpgradeWarning=on
  tms : MATLAB Function  TreatAsAtomicUnit=on
  Qc : Outport
  Pcomp : Outport  Port=2
  Qh : Outport  Port=3
  Ptms : Outport  Port=4
  k_dis : Outport  Port=5
  k_chg : Outport  Port=6
  mc : Outport  Port=7
  mh : Outport  Port=8
  wires:
  Tc/1 -> Mux/1
  Tcs/1 -> Mux/2
  Tpe/1 -> Mux/3
  dT_s/1 -> Mux/4
  tms_en/1 -> Mux/5
  n_mtm/1 -> Mux/6
  en/1 -> Mux/7
  fan_cd/1 -> Mux/8
  fan_pe/1 -> Mux/9
  Mux/1 -> Sample/1
  Sample/1 -> tms/1(u)
  tms/1(y) -> Scan/1
  Scan/1 -> Demux/1
  Demux/1 -> Qc/1
  Demux/2 -> Pcomp/1
  Demux/3 -> Qh/1
  Demux/4 -> Ptms/1
  Demux/5 -> k_dis/1
  Demux/6 -> k_chg/1
  Demux/7 -> mc/1
  Demux/8 -> mh/1

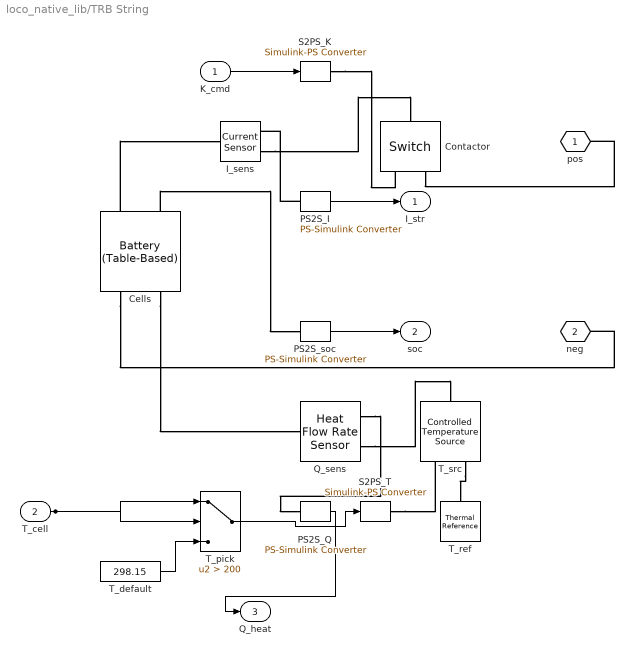
== system loco_native_lib/TRB String ==
  K_cmd : Inport
  T_cell : Inport  Port=2
  Cells : batteryecm_lib/Battery (Table-Based)  SOC_vec=PN.SOC  T_dependence=simscape.enum.tablebattery.temperature_dependence.yes  prm_dir=simscape.enum.tablebattery.prm_dir.noCurrentDirectionality  T_vec=PN.T K  V0_mat=PN.str.V0 V  V0_vec=[3.5057, 3.566, 3.6337, 3.7127, 3.9259, 4.0777, 4.1928] V  V_range=[0 inf] V  R0_mat=PN.str.R0 Ohm  R0_vec=[.0085, .0085, .0087, .0082, .0083, .0085, .0085] Ohm  R0_dis_mat=[.0117, .0085, .009; .011, .0085, .009; .0114, .0087, .0092; .0107, .0082, .0088; .0107, .0083, .0091; .0113, .0085, .0089; .0116, .0085, .0089] Ohm  R0_dis_vec=[.0085, .0085, .0087, .0082, .0083, .0085, .0085] Ohm  R0_ch_mat=[.0117, .0085, .009; .011, .0085, .009; .0114, .0087, .0092; .0107, .0082, .0088; .0107, .0083, .0091; .0113, .0085, .0089; .0116, .0085, .0089] Ohm  R0_ch_vec=[.0085, .0085, .0087, .0082, .0083, .0085, .0085] Ohm  AH=PN.str.Q_Ah A*hr  prm_leak=simscape.enum.tablebattery.prm_leak.disabled  Rleak_vec=[8000, 7000, 6000] Ohm  Rleak=7e3 Ohm  extrapolation_option=simscape.enum.extrapolation.nearest  SOC_port=simscape.enum.tablebattery.enable.yes  prm_dyn=simscape.enum.tablebattery.prm_dyn.rc1  R1_mat=PN.str.R1 Ohm  R1_vec=[.0029, .0024, .0026, .0016, .0023, .0018, .0017] Ohm  tau1_mat=PN.str.tau1 s  tau1_vec=[36, 45, 105, 29, 77, 33, 39] s  R2_mat=[.0109, .0029, .0013; .0069, .0024, .0012; .0047, .0026, .0013; .0034, .0016, .001; .0033, .0023, .0014; .0033, .0018, .0011; .0028, .0017, .0011] Ohm  R2_vec=[.0029, .0024, .0026, .0016, .0023, .0018, .0017] Ohm  tau2_mat=[20, 36, 39; 31, 45, 39; 109, 105, 61; 36, 29, 26; 59, 77, 67; 40, 33, 29; 25, 39, 33] s  tau2_vec=[36, 45, 105, 29, 77, 33, 39] s  R3_mat=[.0109, .0029, .0013; .0069, .0024, .0012; .0047, .0026, .0013; .0034, .0016, .001; .0033, .0023, .0014; .0033, .0018, .0011; .0028, .0017, .0011] Ohm  R3_vec=[.0029, .0024, .0026, .0016, .0023, .0018, .0017] Ohm  tau3_mat=[20, 36, 39; 31, 45, 39; 109, 105, 61; 36, 29, 26; 59, 77, 67; 40, 33, 29; 25, 39, 33] s  tau3_vec=[36, 45, 105, 29, 77, 33, 39] s  R4_mat=[.0109, .0029, .0013; .0069, .0024, .0012; .0047, .0026, .0013; .0034, .0016, .001; .0033, .0023, .0014; .0033, .0018, .0011; .0028, .0017, .0011] Ohm  R4_vec=[.0029, .0024, .0026, .0016, .0023, .0018, .0017] Ohm  tau4_mat=[20, 36, 39; 31, 45, 39; 109, 105, 61; 36, 29, 26; 59, 77, 67; 40, 33, 29; 25, 39, 33] s  tau4_vec=[36, 45, 105, 29, 77, 33, 39] s  R5_mat=[.0109, .0029, .0013; .0069, .0024, .0012; .0047, .0026, .0013; .0034, .0016, .001; .0033, .0023, .0014; .0033, .0018, .0011; .0028, .0017, .0011] Ohm  R5_vec=[.0029, .0024, .0026, .0016, .0023, .0018, .0017] Ohm  tau5_mat=[20, 36, 39; 31, 45, 39; 109, 105, 61; 36, 29, 26; 59, 77, 67; 40, 33, 29; 25, 39, 33] s  tau5_vec=[36, 45, 105, 29, 77, 33, 39] s  prm_fade=simscape.enum.tablebattery.prm_fade.disabled  N0=100  dV0=0  dR0=0  dAH=0  dRleak=0  dR1=0  dR2=0  dR3=0  dR4=0  dR5=0  N0vec=[0, 100, 200, 300]  Tfadevec=[298.15, 323.15] K  dV0vec=[0, 0, 0, 0]  dR0vec=[0, 0, 0, 0]  dAHvec=[0, 0, 0, 0]  dRleakvec=[0, 0, 0, 0]  dR1vec=[0, 0, 0, 0]  dR2vec=[0, 0, 0, 0]  dR3vec=[0, 0, 0, 0]  dR4vec=[0, 0, 0, 0]  dR5vec=[0, 0, 0, 0]  dV0mat=[0, 0; 0, 0; 0, 0; 0, 0]  dR0mat=[0, 0; 0, 0; 0, 0; 0, 0]  dAHmat=[0, 0; 0, 0; 0, 0; 0, 0]  dRleakmat=[0, 0; 0, 0; 0, 0; 0, 0]  dR1mat=[0, 0; 0, 0; 0, 0; 0, 0]  dR2mat=[0, 0; 0, 0; 0, 0; 0, 0]  dR3mat=[0, 0; 0, 0; 0, 0; 0, 0]  dR4mat=[0, 0; 0, 0; 0, 0; 0, 0]  dR5mat=[0, 0; 0, 0; 0, 0; 0, 0]  prm_age_modeling=simscape.enum.tablebattery.prm_age_modeling.equation  storage_dt_age_vec=[0] d  storage_T_age_vec=[273] K  prm_age_OCV=simscape.enum.tablebattery.prm_age_OCV.OCV  OCV_age=0.9  SOC_age=0.6  prm_age_resistance=simscape.enum.tablebattery.prm_age.disabled  OCV_scaling_age_resistance=2.2134e6  OCV_offset_age_resistance=1.632e6  temp_exp_age_resistance=0.515833569 V  t_exp_age_resistance=0.75  T_age_vec_resistance=[273.15, 298.15, 323.15] K  dt_age_vec_resistance=[0, 90, 180, 270] d  dR0_age_vec=[0, 0, 0]  t_meas_dR0_age=100 d  dR0_age_mat=[0, 0, 0; 0, 0, 0; 0, 0, 0; 0, 0, 0]  prm_age_capacity=simscape.enum.tablebattery.prm_age.disabled  OCV_scaling_age_capacity=1.5097e07  OCV_offset_age_capacity=8.3625e06  temp_exp_age_capacity=0.6011 V  t_exp_age_capacity=0.75  T_age_vec_capacity=[273.15, 298.15, 323.15] K  dt_age_vec_capacity=[0, 90, 180, 270] d  dAH_age_vec=[0, 0, 0]  t_meas_dAH_age=100 d  dAH_age_mat=[0, 0, 0; 0, 0, 0; 0, 0, 0; 0, 0, 0]  thermal_port=simscape.enum.thermaleffects.model  temperature=298.15 K  thermal_mass=100 J/K  i_specify=off  i_priority=None  i=0 A  i_nominal_specify=off  i_nominal_value=1  i_nominal_unit=A  v_specify=off  v_priority=None  v=0 V  v_nominal_specify=off  v_nominal_value=1  v_nominal_unit=V  stateOfCharge_specify=on  stateOfCharge_priority=High  stateOfCharge=PN.str.soc0  stateOfCharge_nominal_specify=off  stateOfCharge_nominal_value=1  stateOfCharge_nominal_unit=1  num_cycles_specify=off  num_cycles_priority=High  num_cycles=0  num_cycles_nominal_specify=off  num_cycles_nominal_value=1  num_cycles_nominal_unit=1  cell_temperature_specify=on  cell_temperature_priority=Low  cell_temperature=298.15 K  cell_temperature_nominal_specify=off  cell_temperature_nominal_value=1  cell_temperature_nominal_unit=K
  Contactor : fl_lib/Electrical/Electrical Elements/Switch  R_closed=0.1e-3 Ohm  G_open=1e-9 1/Ohm  Threshold=0.5  i_specify=off  i_priority=None  i=0 A  i_nominal_specify=off  i_nominal_value=1  i_nominal_unit=A  v_specify=off  v_priority=None  v=0 V  v_nominal_specify=off  v_nominal_value=1  v_nominal_unit=V
  I_sens : fl_lib/Electrical/Electrical Sensors/Current Sensor
  PS2S_I : nesl_utility/PS-Simulink Converter  PhysicalDomain=network_engine_domain  SubClassName=ps_output  LeftPortType=input  RightPortType=output  PseudoPeriodic=off  Frequencies=[]  VectorFormat=inherit  Unit=A  AffineConversion=off
  PS2S_Q : nesl_utility/PS-Simulink Converter  PhysicalDomain=network_engine_domain  SubClassName=ps_output  LeftPortType=input  RightPortType=output  PseudoPeriodic=off  Frequencies=[]  VectorFormat=inherit  Unit=W  AffineConversion=off
  PS2S_soc : nesl_utility/PS-Simulink Converter  PhysicalDomain=network_engine_domain  SubClassName=ps_output  LeftPortType=input  RightPortType=output  PseudoPeriodic=off  Frequencies=[]  VectorFormat=inherit  Unit=1  AffineConversion=off
  Q_sens : fl_lib/Thermal/Thermal Sensors/Heat Flow Rate Sensor
  S2PS_K : nesl_utility/Simulink-PS Converter  PhysicalDomain=network_engine_domain  SubClassName=ps_input  LeftPortType=input  RightPortType=output  PseudoPeriodic=off  Frequencies=[]  NoiseDistribution=none  NoiseParameters=[]  Unit=1  AffineConversion=off  FilteringAndDerivatives=provide  SimscapeFilterOrder=1  InputFilterTimeConstant=0.001  UdotUserProvided=0
  S2PS_T : nesl_utility/Simulink-PS Converter  PhysicalDomain=network_engine_domain  SubClassName=ps_input  LeftPortType=input  RightPortType=output  PseudoPeriodic=off  Frequencies=[]  NoiseDistribution=none  NoiseParameters=[]  Unit=K  AffineConversion=off  FilteringAndDerivatives=filter  SimscapeFilterOrder=1  InputFilterTimeConstant=1  UdotUserProvided=0
  T_default : Constant  Value=298.15
  T_pick : Switch  Criteria=u2 > Threshold  Threshold=200  SaturateOnIntegerOverflow=off  InputSameDT=off
  T_ref : fl_lib/Thermal/Thermal Elements/Thermal Reference
  T_src : fl_lib/Thermal/Thermal Sources/Controlled Temperature Source
  pos : PMIOPort  Side=Right
  neg : PMIOPort  Port=2  Side=Right
  I_str : Outport
  soc : Outport  Port=2
  Q_heat : Outport  Port=3
  wires:
  K_cmd/1 -> S2PS_K/1
  PS2S_I/1 -> I_str/1
  PS2S_soc/1 -> soc/1
  T_cell/1 -> T_pick/1, T_pick/2
  T_default/1 -> T_pick/3
  T_pick/1 -> S2PS_T/1
  PS2S_Q/1 -> Q_heat/1
  connections:
  Cells/LConn1 -- I_sens/LConn1
  PS2S_I/LConn1 -- I_sens/RConn1
  I_sens/RConn2 -- Contactor/LConn1
  Contactor/RConn2 -- pos/RConn1
  Cells/RConn1 -- neg/RConn1
  S2PS_K/RConn1 -- Contactor/RConn1
  Cells/LConn2 -- PS2S_soc/LConn1
  Cells/RConn2 -- Q_sens/LConn1
  Q_sens/RConn2 -- T_src/LConn1
  T_src/RConn2 -- T_ref/LConn1
  S2PS_T/RConn1 -- T_src/RConn1
  Q_sens/RConn1 -- PS2S_Q/LConn1
